simulink model "TrafficLightModel"  (R2026a)
settings: Solver=VariableStepAuto  StopTime=60
StartFcn:
  | learning.simulink.modelCallbacks.startFunction(gcs);
StopFcn:
  | learning.simulink.modelCallbacks.stopFunction(gcs);
model workspace (MAT data in the model file):
  courseObject.course = 'stateflow'
  courseObject.chapter = 3
  courseObject.lesson = 3
  courseObject.section = 1
  courseObject.task = 1
CloseFcn:
  | learning.simulink.cleanupOnlineTraining;learning.simulink.Application.getInstance().dduxLogMatlabEvent("ModelClosed");
Description:
  | TrainingCourseModel
settings Model: Creator=PC  LastModifiedBy=PC

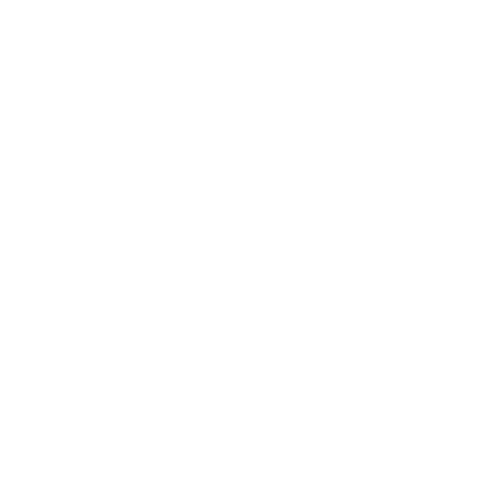
[thumbnail: Simulink's stored preview of the top-level diagram]
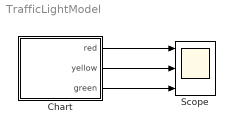
== system TrafficLightModel ==
  Chart : Stateflow chart  TreatAsAtomicUnit=on
  Scope : Scope  NumInputPorts=3
      settings: ActiveDisplayYMinimum=-0.125  ActiveDisplayYMaximum=1.125
  wires:
  Chart/3(green) -> Scope/3
  Chart/1(red) -> Scope/1
  Chart/2(yellow) -> Scope/2

== stateflow chart TrafficLightModel/Chart ==
  state Stop
    entry:
    red = 1;
    yellow = 0;
    green = 0;
  state PrepareToStop
    entry:
    red = 0;
    yellow = 1;
    green = 0;
  state Go
    entry:
    red = 0;
    yellow = 0;
    green = 1;
  (default) -> Stop
  Stop -> (junction 9)
  (junction 9) -> (junction 8) : after(3,sec)
  PrepareToStop -> Stop : after(3,sec)
  Go -> PrepareToStop : after(10,sec)
  (junction 8) -> Go
  data: red output; yellow output; green output
